simulink model "EV_Bus_Forward"  (R2025a)
settings: Solver=ode23t  StartTime=0.0  StopTime=CaseStopTime  MaxStep=Comp.MaxStep  RelTol=1e-5  AbsTol=1e-7
model workspace (MAT data in the model file):
  CaseStopTime = 300
  Comp : object (value not decoded)
  MeasuredForceBias = 1114.3044183
  MeasuredTraction = [0 0.01 0.02 0.03 0.04 0.05 0.06 0.07 0.08 0.09 0.1 0.11 ... (60002 elements, 30001x2)]
  P : object (value not decoded)
  SignalNames : object (value not decoded)
  SlopeProfile = [0 85 100 140 155 180 200 300 0 0 4 4 ... (16 elements, 8x2)]
  SpeedProfile = [0 5 25 55 70 85 105 140 160 180 200 225 ... (32 elements, 16x2)]
  TemperatureProfile = [0  25; 150  30; 300  35]
values from neighbouring files (symbols this model uses):
  Comp = struct('Tau',baseTau,'Limit',min(0.03*P.Mass*P.Gravity,0.25*driveForce),      'InitialForce',0,'Enable',1,'MinAdaptSpeed',opt(options,'MinAdaptSpeed_mps',0.5),      'MeasurementStart',0,'MeasurementEnd',duration)    [run_EV_Bus_case.m]
  P = getVariable(mw,'P')    [run_EV_Bus_case.m]
(part 2 of 2)

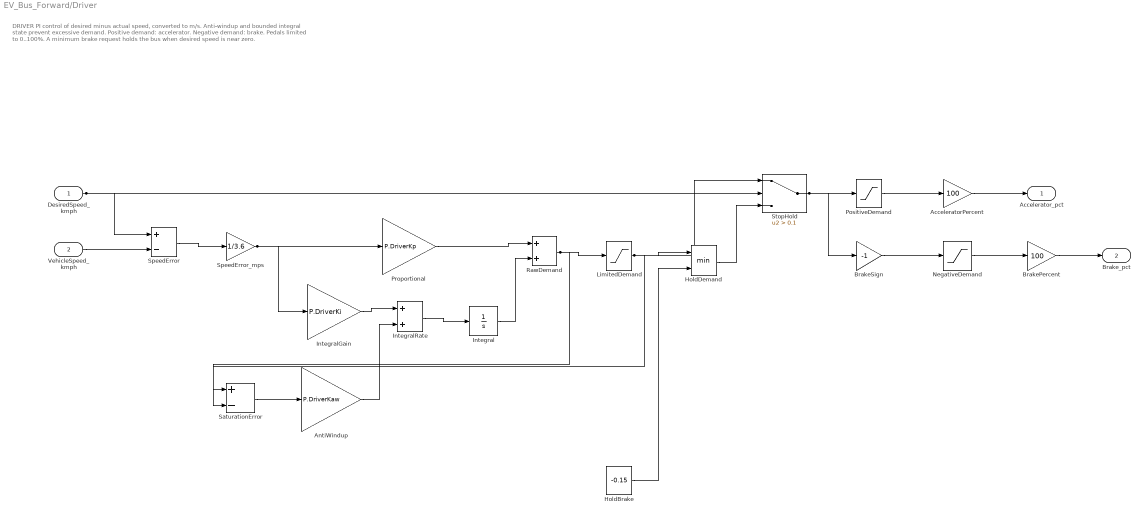
== system EV_Bus_Forward/Driver ==
  note: DRIVER
      | PI control of desired minus actual speed, converted to m/s.
      | Anti-windup and bounded integral state prevent excessive demand.
      | Positive demand: accelerator. Negative demand: brake. Pedals limited to 0..100%.
      | A minimum brake request holds the bus when desired speed is near zero.
  DesiredSpeed_kmph : Inport
  VehicleSpeed_kmph : Inport  Port=2
  AcceleratorPercent : Gain  Gain=100
  AntiWindup : Gain  Gain=P.DriverKaw
  BrakePercent : Gain  Gain=100
  BrakeSign : Gain  Gain=-1
  HoldBrake : Constant  Value=-0.15
  HoldDemand : MinMax  Inputs=2
  Integral : Integrator  LimitOutput=on  UpperSaturationLimit=0.6  LowerSaturationLimit=-0.6
  IntegralGain : Gain  Gain=P.DriverKi
  IntegralRate : Sum
  LimitedDemand : Saturate  UpperLimit=1  LowerLimit=-1
  NegativeDemand : Saturate  UpperLimit=1  LowerLimit=0
  PositiveDemand : Saturate  UpperLimit=1  LowerLimit=0
  Proportional : Gain  Gain=P.DriverKp
  RawDemand : Sum
  SaturationError : Sum  Inputs=+-
  SpeedError : Sum  Inputs=+-
  SpeedError_mps : Gain  Gain=1/3.6
  StopHold : Switch  Criteria=u2 > Threshold  Threshold=0.1  SaturateOnIntegerOverflow=off  InputSameDT=off
  Accelerator_pct : Outport
  Brake_pct : Outport  Port=2
  wires:
  AntiWindup/1 -> IntegralRate/2
  DesiredSpeed_kmph/1 -> StopHold/2, SpeedError/1
  VehicleSpeed_kmph/1 -> SpeedError/2
  RawDemand/1 -> SaturationError/2, LimitedDemand/1
  SaturationError/1 -> AntiWindup/1
  SpeedError_mps/1 -> Proportional/1, IntegralGain/1
  NegativeDemand/1 -> BrakePercent/1
  StopHold/1 -> PositiveDemand/1, BrakeSign/1
  IntegralRate/1 -> Integral/1
  SpeedError/1 -> SpeedError_mps/1
  Proportional/1 -> RawDemand/1
  IntegralGain/1 -> IntegralRate/1
  Integral/1 -> RawDemand/2
  LimitedDemand/1 -> SaturationError/1, StopHold/1, HoldDemand/1
  HoldBrake/1 -> HoldDemand/2
  HoldDemand/1 -> StopHold/3
  PositiveDemand/1 -> AcceleratorPercent/1
  BrakeSign/1 -> NegativeDemand/1
  AcceleratorPercent/1 -> Accelerator_pct/1
  BrakePercent/1 -> Brake_pct/1

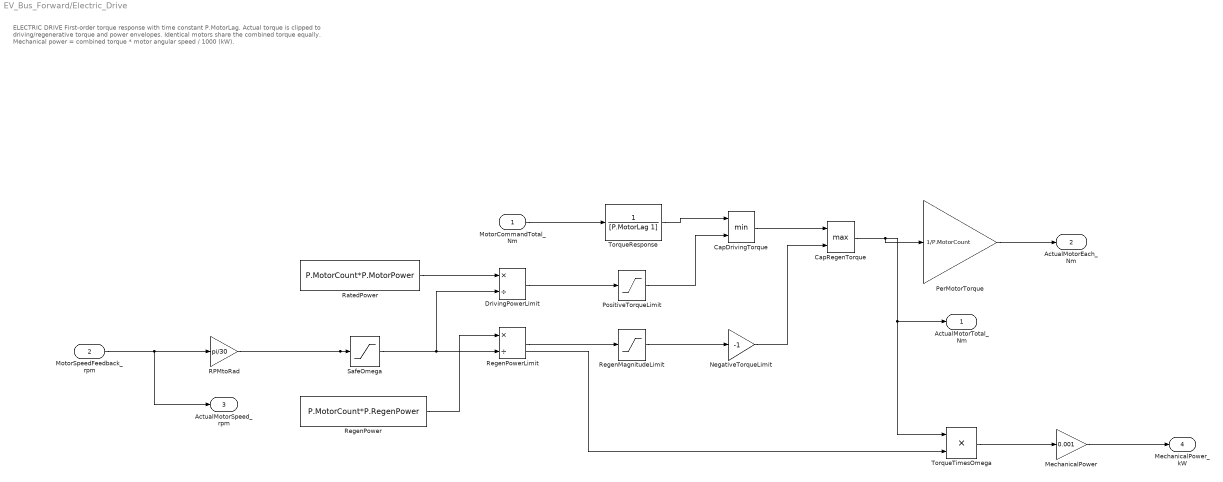
== system EV_Bus_Forward/Electric_Drive ==
  note: ELECTRIC DRIVE
      | First-order torque response with time constant P.MotorLag.
      | Actual torque is clipped to driving/regenerative torque and power envelopes.
      | Identical motors share the combined torque equally.
      | Mechanical power = combined torque * motor angular speed / 1000 (kW).
  MotorCommandTotal_Nm : Inport
  MotorSpeedFeedback_rpm : Inport  Port=2
  CapDrivingTorque : MinMax  Inputs=2
  CapRegenTorque : MinMax  Function=max  Inputs=2
  DrivingPowerLimit : Product  Inputs=*/
  MechanicalPower : Gain  Gain=0.001
  NegativeTorqueLimit : Gain  Gain=-1
  PerMotorTorque : Gain  Gain=1/P.MotorCount
  PositiveTorqueLimit : Saturate  UpperLimit=P.MotorCount*P.MotorPeakTorque  LowerLimit=0
  RPMtoRad : Gain  Gain=pi/30
  RatedPower : Constant  Value=P.MotorCount*P.MotorPower
  RegenMagnitudeLimit : Saturate  UpperLimit=P.MotorCount*P.RegenPeakTorque  LowerLimit=0
  RegenPower : Constant  Value=P.MotorCount*P.RegenPower
  RegenPowerLimit : Product  Inputs=*/
  SafeOmega : Saturate  UpperLimit=inf  LowerLimit=1
  TorqueResponse : TransferFcn  Denominator=[P.MotorLag 1]
  TorqueTimesOmega : Product  Inputs=**
  ActualMotorTotal_Nm : Outport
  ActualMotorEach_Nm : Outport  Port=2
  ActualMotorSpeed_rpm : Outport  Port=3
  MechanicalPower_kW : Outport  Port=4
  wires:
  MotorCommandTotal_Nm/1 -> TorqueResponse/1
  SafeOmega/1 -> RegenPowerLimit/2, DrivingPowerLimit/2
  MotorSpeedFeedback_rpm/1 -> ActualMotorSpeed_rpm/1, RPMtoRad/1
  RegenPower/1 -> RegenPowerLimit/1
  RegenPowerLimit/1 -> RegenMagnitudeLimit/1
  DrivingPowerLimit/1 -> PositiveTorqueLimit/1
  RatedPower/1 -> DrivingPowerLimit/1
  RPMtoRad/1 -> TorqueTimesOmega/2, SafeOmega/1
  TorqueTimesOmega/1 -> MechanicalPower/1
  TorqueResponse/1 -> CapDrivingTorque/1
  RegenMagnitudeLimit/1 -> NegativeTorqueLimit/1
  PositiveTorqueLimit/1 -> CapDrivingTorque/2
  CapDrivingTorque/1 -> CapRegenTorque/1
  NegativeTorqueLimit/1 -> CapRegenTorque/2
  MechanicalPower/1 -> MechanicalPower_kW/1
  CapRegenTorque/1 -> TorqueTimesOmega/1, ActualMotorTotal_Nm/1, PerMotorTorque/1
  PerMotorTorque/1 -> ActualMotorEach_Nm/1

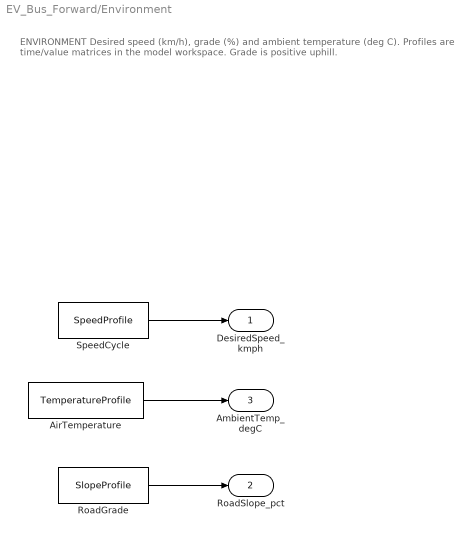
== system EV_Bus_Forward/Environment ==
  note: ENVIRONMENT
      | Desired speed (km/h), grade (%) and ambient temperature (deg C).
      | Profiles are time/value matrices in the model workspace. Grade is positive uphill.
  AirTemperature : FromWorkspace  VariableName=TemperatureProfile
  RoadGrade : FromWorkspace  VariableName=SlopeProfile
  SpeedCycle : FromWorkspace  VariableName=SpeedProfile
  DesiredSpeed_kmph : Outport
  RoadSlope_pct : Outport  Port=2
  AmbientTemp_degC : Outport  Port=3
  wires:
  RoadGrade/1 -> RoadSlope_pct/1
  AirTemperature/1 -> AmbientTemp_degC/1
  SpeedCycle/1 -> DesiredSpeed_kmph/1

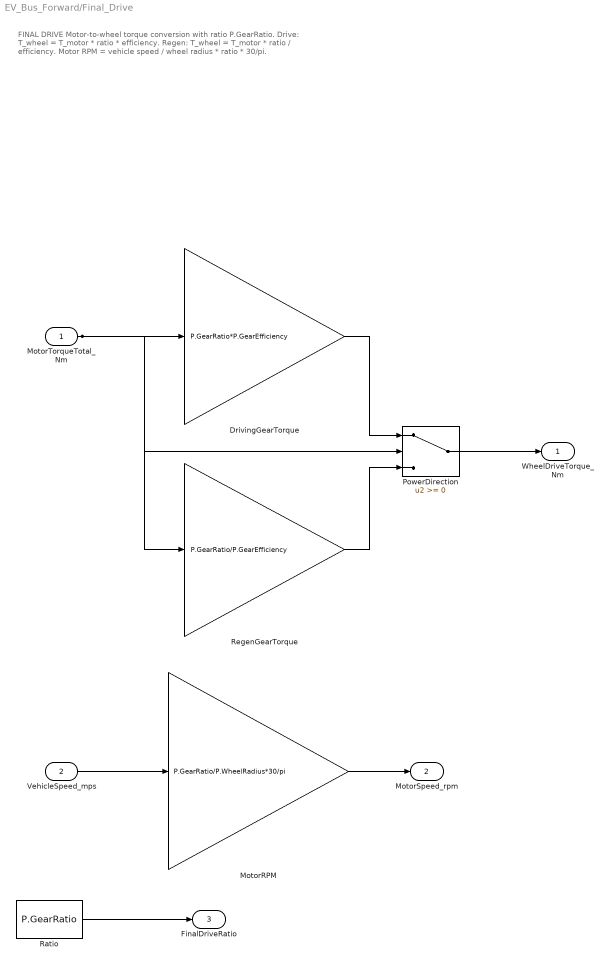
== system EV_Bus_Forward/Final_Drive ==
  note: FINAL DRIVE
      | Motor-to-wheel torque conversion with ratio P.GearRatio.
      | Drive: T_wheel = T_motor * ratio * efficiency.
      | Regen: T_wheel = T_motor * ratio / efficiency.
      | Motor RPM = vehicle speed / wheel radius * ratio * 30/pi.
  MotorTorqueTotal_Nm : Inport
  VehicleSpeed_mps : Inport  Port=2
  DrivingGearTorque : Gain  Gain=P.GearRatio*P.GearEfficiency
  MotorRPM : Gain  Gain=P.GearRatio/P.WheelRadius*30/pi
  PowerDirection : Switch  SaturateOnIntegerOverflow=off  InputSameDT=off
  Ratio : Constant  Value=P.GearRatio
  RegenGearTorque : Gain  Gain=P.GearRatio/P.GearEfficiency
  WheelDriveTorque_Nm : Outport
  MotorSpeed_rpm : Outport  Port=2
  FinalDriveRatio : Outport  Port=3
  wires:
  MotorTorqueTotal_Nm/1 -> PowerDirection/2, RegenGearTorque/1, DrivingGearTorque/1
  PowerDirection/1 -> WheelDriveTorque_Nm/1
  MotorRPM/1 -> MotorSpeed_rpm/1
  RegenGearTorque/1 -> PowerDirection/3
  DrivingGearTorque/1 -> PowerDirection/1
  Ratio/1 -> FinalDriveRatio/1
  VehicleSpeed_mps/1 -> MotorRPM/1

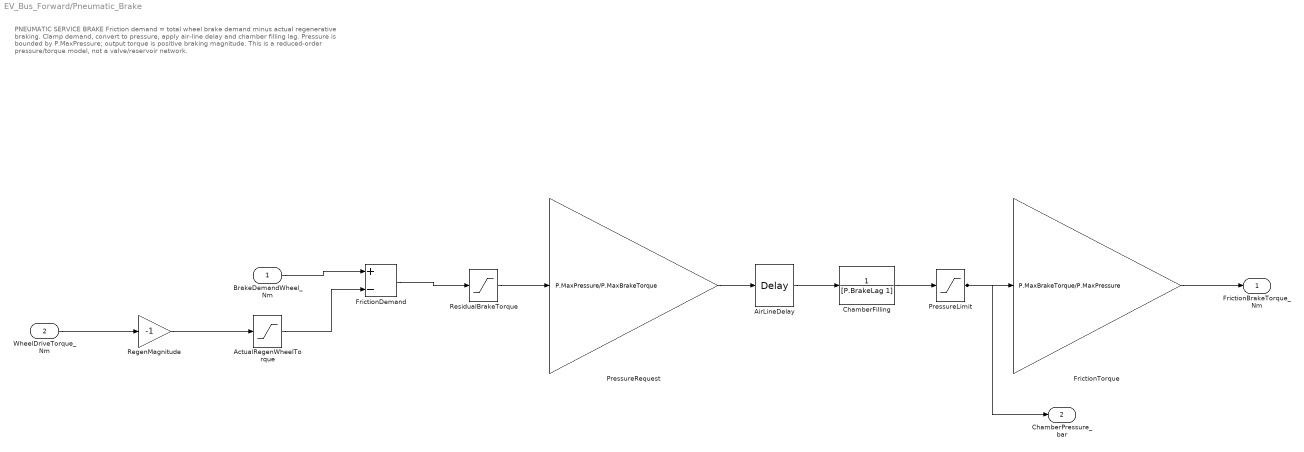
== system EV_Bus_Forward/Pneumatic_Brake ==
  note: PNEUMATIC SERVICE BRAKE
      | Friction demand = total wheel brake demand minus actual regenerative braking.
      | Clamp demand, convert to pressure, apply air-line delay and chamber filling lag.
      | Pressure is bounded by P.MaxPressure; output torque is positive braking magnitude.
      | This is a reduced-order pressure/torque model, not a valve/reservoir network.
  BrakeDemandWheel_Nm : Inport
  WheelDriveTorque_Nm : Inport  Port=2
  ActualRegenWheelTorque : Saturate  UpperLimit=inf  LowerLimit=0
  AirLineDelay : TransportDelay  DelayTime=P.BrakeDelay
  ChamberFilling : TransferFcn  Denominator=[P.BrakeLag 1]
  FrictionDemand : Sum  Inputs=+-
  FrictionTorque : Gain  Gain=P.MaxBrakeTorque/P.MaxPressure
  PressureLimit : Saturate  UpperLimit=P.MaxPressure  LowerLimit=0
  PressureRequest : Gain  Gain=P.MaxPressure/P.MaxBrakeTorque
  RegenMagnitude : Gain  Gain=-1
  ResidualBrakeTorque : Saturate  UpperLimit=P.MaxBrakeTorque  LowerLimit=0
  FrictionBrakeTorque_Nm : Outport
  ChamberPressure_bar : Outport  Port=2
  wires:
  BrakeDemandWheel_Nm/1 -> FrictionDemand/1
  AirLineDelay/1 -> ChamberFilling/1
  FrictionDemand/1 -> ResidualBrakeTorque/1
  PressureLimit/1 -> ChamberPressure_bar/1, FrictionTorque/1
  ActualRegenWheelTorque/1 -> FrictionDemand/2
  FrictionTorque/1 -> FrictionBrakeTorque_Nm/1
  WheelDriveTorque_Nm/1 -> RegenMagnitude/1
  PressureRequest/1 -> AirLineDelay/1
  ResidualBrakeTorque/1 -> PressureRequest/1
  RegenMagnitude/1 -> ActualRegenWheelTorque/1
  ChamberFilling/1 -> PressureLimit/1

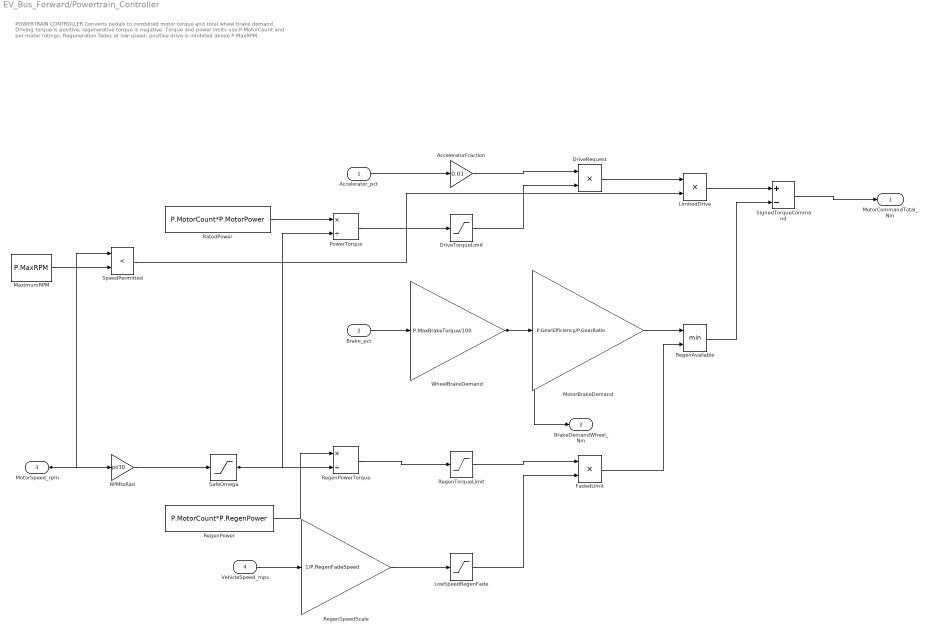
== system EV_Bus_Forward/Powertrain_Controller ==
  note: POWERTRAIN CONTROLLER
      | Converts pedals to combined motor torque and total wheel brake demand.
      | Driving torque is positive; regenerative torque is negative.
      | Torque and power limits use P.MotorCount and per-motor ratings.
      | Regeneration fades at low speed; positive drive is inhibited above P.MaxRPM.
  Accelerator_pct : Inport
  Brake_pct : Inport  Port=2
  MotorSpeed_rpm : Inport  Port=3
  VehicleSpeed_mps : Inport  Port=4
  AcceleratorFraction : Gain  Gain=0.01
  DriveRequest : Product  Inputs=**
  DriveTorqueLimit : Saturate  UpperLimit=P.MotorCount*P.MotorPeakTorque  LowerLimit=0
  FadedLimit : Product  Inputs=**
  LimitedDrive : Product  Inputs=**
  LowSpeedRegenFade : Saturate  UpperLimit=1  LowerLimit=0
  MaximumRPM : Constant  Value=P.MaxRPM
  MotorBrakeDemand : Gain  Gain=P.GearEfficiency/P.GearRatio
  PowerTorque : Product  Inputs=*/
  RPMtoRad : Gain  Gain=pi/30
  RatedPower : Constant  Value=P.MotorCount*P.MotorPower
  RegenAvailable : MinMax  Inputs=2
  RegenPower : Constant  Value=P.MotorCount*P.RegenPower
  RegenPowerTorque : Product  Inputs=*/
  RegenSpeedScale : Gain  Gain=1/P.RegenFadeSpeed
  RegenTorqueLimit : Saturate  UpperLimit=P.MotorCount*P.RegenPeakTorque  LowerLimit=0
  SafeOmega : Saturate  UpperLimit=inf  LowerLimit=1
  SignedTorqueCommand : Sum  Inputs=+-
  SpeedPermitted : RelationalOperator  Operator=<  OutDataTypeStr=boolean  RndMeth=Simplest  InputSameDT=off
  WheelBrakeDemand : Gain  Gain=P.MaxBrakeTorque/100
  MotorCommandTotal_Nm : Outport
  BrakeDemandWheel_Nm : Outport  Port=2
  wires:
  VehicleSpeed_mps/1 -> RegenSpeedScale/1
  FadedLimit/1 -> RegenAvailable/2
  MotorSpeed_rpm/1 -> SpeedPermitted/1, RPMtoRad/1
  DriveRequest/1 -> LimitedDrive/1
  MaximumRPM/1 -> SpeedPermitted/2
  SpeedPermitted/1 -> LimitedDrive/2
  RPMtoRad/1 -> SafeOmega/1
  RegenPower/1 -> RegenPowerTorque/1
  RegenAvailable/1 -> SignedTorqueCommand/2
  PowerTorque/1 -> DriveTorqueLimit/1
  SafeOmega/1 -> RegenPowerTorque/2, PowerTorque/2
  RegenTorqueLimit/1 -> FadedLimit/1
  RatedPower/1 -> PowerTorque/1
  LimitedDrive/1 -> SignedTorqueCommand/1
  DriveTorqueLimit/1 -> DriveRequest/2
  Accelerator_pct/1 -> AcceleratorFraction/1
  Brake_pct/1 -> WheelBrakeDemand/1
  RegenPowerTorque/1 -> RegenTorqueLimit/1
  RegenSpeedScale/1 -> LowSpeedRegenFade/1
  AcceleratorFraction/1 -> DriveRequest/1
  WheelBrakeDemand/1 -> BrakeDemandWheel_Nm/1, MotorBrakeDemand/1
  LowSpeedRegenFade/1 -> FadedLimit/2
  MotorBrakeDemand/1 -> RegenAvailable/1
  SignedTorqueCommand/1 -> MotorCommandTotal_Nm/1

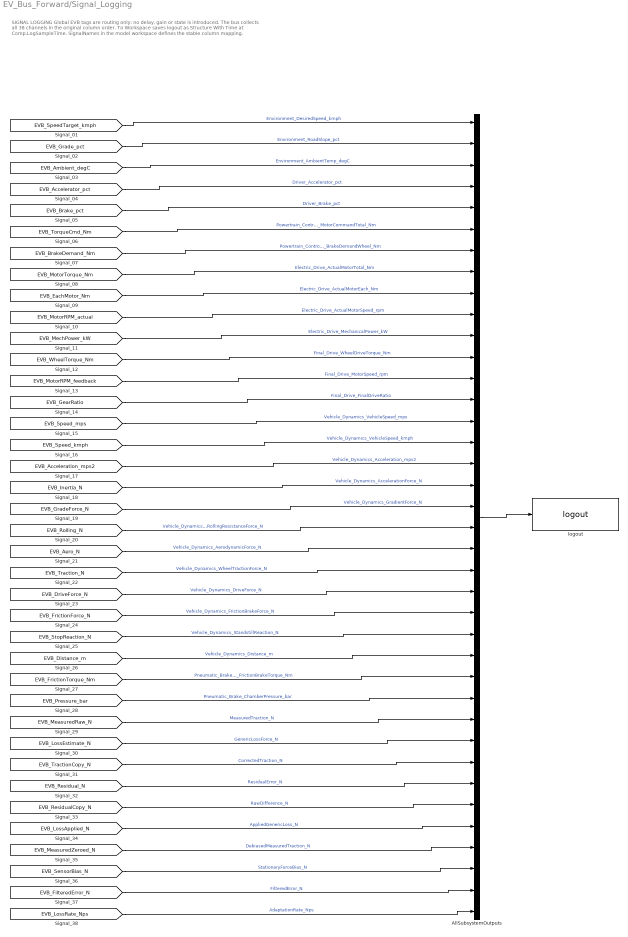
== system EV_Bus_Forward/Signal_Logging ==
  note: SIGNAL LOGGING
      | Global EVB tags are routing only: no delay, gain or state is introduced.
      | The bus collects all 38 channels in the original column order.
      | To Workspace saves logout as Structure With Time at Comp.LogSampleTime.
      | SignalNames in the model workspace defines the stable column mapping.
  AllSubsystemOutputs : BusCreator  Inputs=38
  logout : ToWorkspace  VariableName=logout  SaveFormat=Structure With Time  SampleTime=Comp.LogSampleTime
  wires:
  [EVB_LossRate_Nps] -> AllSubsystemOutputs/38  "AdaptationRate_Nps"
  [EVB_FilteredError_N] -> AllSubsystemOutputs/37  "FilteredError_N"
  [EVB_SensorBias_N] -> AllSubsystemOutputs/36  "StationaryForceBias_N"
  [EVB_MeasuredZeroed_N] -> AllSubsystemOutputs/35  "DebiasedMeasuredTraction_N"
  [EVB_LossApplied_N] -> AllSubsystemOutputs/34  "AppliedGenericLoss_N"
  [EVB_ResidualCopy_N] -> AllSubsystemOutputs/33  "RawDifference_N"
  [EVB_Residual_N] -> AllSubsystemOutputs/32  "ResidualError_N"
  [EVB_TractionCopy_N] -> AllSubsystemOutputs/31  "CorrectedTraction_N"
  [EVB_LossEstimate_N] -> AllSubsystemOutputs/30  "GenericLossForce_N"
  [EVB_MeasuredRaw_N] -> AllSubsystemOutputs/29  "MeasuredTraction_N"
  [EVB_Pressure_bar] -> AllSubsystemOutputs/28  "Pneumatic_Brake_ChamberPressure_bar"
  [EVB_FrictionTorque_Nm] -> AllSubsystemOutputs/27  "Pneumatic_Brake_FrictionBrakeTorque_Nm"
  [EVB_Distance_m] -> AllSubsystemOutputs/26  "Vehicle_Dynamics_Distance_m"
  [EVB_StopReaction_N] -> AllSubsystemOutputs/25  "Vehicle_Dynamics_StandstillReaction_N"
  [EVB_FrictionForce_N] -> AllSubsystemOutputs/24  "Vehicle_Dynamics_FrictionBrakeForce_N"
  [EVB_DriveForce_N] -> AllSubsystemOutputs/23  "Vehicle_Dynamics_DriveForce_N"
  [EVB_Traction_N] -> AllSubsystemOutputs/22  "Vehicle_Dynamics_WheelTractionForce_N"
  [EVB_Aero_N] -> AllSubsystemOutputs/21  "Vehicle_Dynamics_AerodynamicForce_N"
  [EVB_Rolling_N] -> AllSubsystemOutputs/20  "Vehicle_Dynamics_RollingResistanceForce_N"
  [EVB_GradeForce_N] -> AllSubsystemOutputs/19  "Vehicle_Dynamics_GradientForce_N"
  [EVB_Inertia_N] -> AllSubsystemOutputs/18  "Vehicle_Dynamics_AccelerationForce_N"
  [EVB_Acceleration_mps2] -> AllSubsystemOutputs/17  "Vehicle_Dynamics_Acceleration_mps2"
  [EVB_Speed_kmph] -> AllSubsystemOutputs/16  "Vehicle_Dynamics_VehicleSpeed_kmph"
  [EVB_Speed_mps] -> AllSubsystemOutputs/15  "Vehicle_Dynamics_VehicleSpeed_mps"
  [EVB_GearRatio] -> AllSubsystemOutputs/14  "Final_Drive_FinalDriveRatio"
  [EVB_MotorRPM_feedback] -> AllSubsystemOutputs/13  "Final_Drive_MotorSpeed_rpm"
  [EVB_WheelTorque_Nm] -> AllSubsystemOutputs/12  "Final_Drive_WheelDriveTorque_Nm"
  [EVB_MechPower_kW] -> AllSubsystemOutputs/11  "Electric_Drive_MechanicalPower_kW"
  [EVB_MotorRPM_actual] -> AllSubsystemOutputs/10  "Electric_Drive_ActualMotorSpeed_rpm"
  [EVB_EachMotor_Nm] -> AllSubsystemOutputs/9  "Electric_Drive_ActualMotorEach_Nm"
  [EVB_MotorTorque_Nm] -> AllSubsystemOutputs/8  "Electric_Drive_ActualMotorTotal_Nm"
  [EVB_BrakeDemand_Nm] -> AllSubsystemOutputs/7  "Powertrain_Controller_BrakeDemandWheel_Nm"
  [EVB_TorqueCmd_Nm] -> AllSubsystemOutputs/6  "Powertrain_Controller_MotorCommandTotal_Nm"
  [EVB_Brake_pct] -> AllSubsystemOutputs/5  "Driver_Brake_pct"
  [EVB_Accelerator_pct] -> AllSubsystemOutputs/4  "Driver_Accelerator_pct"
  [EVB_Ambient_degC] -> AllSubsystemOutputs/3  "Environment_AmbientTemp_degC"
  [EVB_Grade_pct] -> AllSubsystemOutputs/2  "Environment_RoadSlope_pct"
  [EVB_SpeedTarget_kmph] -> AllSubsystemOutputs/1  "Environment_DesiredSpeed_kmph"
  AllSubsystemOutputs/1 -> logout/1

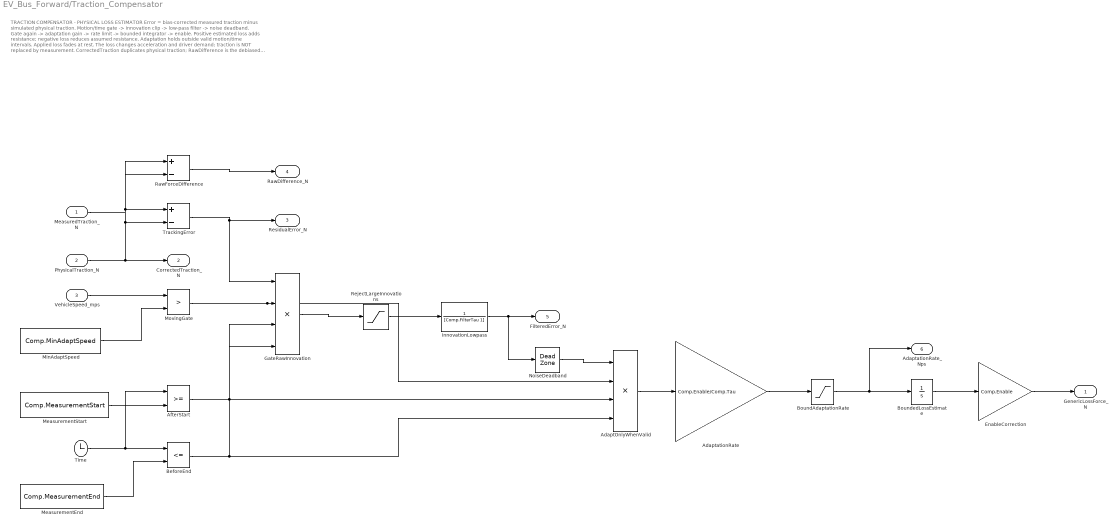
== system EV_Bus_Forward/Traction_Compensator ==
  note: TRACTION COMPENSATOR - PHYSICAL LOSS ESTIMATOR
      | Error = bias-corrected measured traction minus simulated physical traction.
      | Motion/time gate -> innovation clip -> low-pass filter -> noise deadband.
      | Gate again -> adaptation gain -> rate limit -> bounded integrator -> enable.
      | Positive estimated loss adds resistance; negative loss reduces assumed resistance.
      | Adaptation holds outside valid motion/time intervals. Applied loss fades at rest.
      | The loss changes acceleration and driver demand; traction is NOT replaced by measurement.
      | CorrectedTraction duplicates physical traction; RawDifference is the debiased residual.
  MeasuredTraction_N : Inport
  PhysicalTraction_N : Inport  Port=2
  VehicleSpeed_mps : Inport  Port=3
  AdaptOnlyWhenValid : Product  Inputs=****
  AdaptationRate : Gain  Gain=Comp.Enable/Comp.Tau
  AfterStart : RelationalOperator  OutDataTypeStr=boolean  RndMeth=Simplest  InputSameDT=off
  BeforeEnd : RelationalOperator  Operator=<=  OutDataTypeStr=boolean  RndMeth=Simplest  InputSameDT=off
  BoundAdaptationRate : Saturate  UpperLimit=Comp.MaxRate  LowerLimit=-Comp.MaxRate
  BoundedLossEstimate : Integrator  InitialCondition=Comp.InitialForce  LimitOutput=on  UpperSaturationLimit=Comp.Limit  LowerSaturationLimit=-Comp.Limit
  EnableCorrection : Gain  Gain=Comp.Enable
  GateRawInnovation : Product  Inputs=****
  InnovationLowpass : TransferFcn  Denominator=[Comp.FilterTau 1]
  MeasurementEnd : Constant  Value=Comp.MeasurementEnd
  MeasurementStart : Constant  Value=Comp.MeasurementStart
  MinAdaptSpeed : Constant  Value=Comp.MinAdaptSpeed
  MovingGate : RelationalOperator  Operator=>  OutDataTypeStr=boolean  RndMeth=Simplest  InputSameDT=off
  NoiseDeadband : DeadZone  LowerValue=-Comp.Deadband  UpperValue=Comp.Deadband
  RawForceDifference : Sum  Inputs=+-
  RejectLargeInnovations : Saturate  UpperLimit=Comp.ErrorClip  LowerLimit=-Comp.ErrorClip
  Time : Clock
  TrackingError : Sum  Inputs=+-
  GenericLossForce_N : Outport
  CorrectedTraction_N : Outport  Port=2
  ResidualError_N : Outport  Port=3
  RawDifference_N : Outport  Port=4
  FilteredError_N : Outport  Port=5
  AdaptationRate_Nps : Outport  Port=6
  wires:
  PhysicalTraction_N/1 -> RawForceDifference/2, TrackingError/2, CorrectedTraction_N/1
  MeasuredTraction_N/1 -> RawForceDifference/1, TrackingError/1
  VehicleSpeed_mps/1 -> MovingGate/1
  RawForceDifference/1 -> RawDifference_N/1
  MovingGate/1 -> AdaptOnlyWhenValid/2, GateRawInnovation/2
  TrackingError/1 -> GateRawInnovation/1, ResidualError_N/1
  MeasurementEnd/1 -> BeforeEnd/2
  MinAdaptSpeed/1 -> MovingGate/2
  Time/1 -> BeforeEnd/1, AfterStart/1
  RejectLargeInnovations/1 -> InnovationLowpass/1
  MeasurementStart/1 -> AfterStart/2
  AfterStart/1 -> AdaptOnlyWhenValid/3, GateRawInnovation/3
  AdaptationRate/1 -> BoundAdaptationRate/1
  BeforeEnd/1 -> GateRawInnovation/4, AdaptOnlyWhenValid/4
  GateRawInnovation/1 -> RejectLargeInnovations/1
  InnovationLowpass/1 -> NoiseDeadband/1, FilteredError_N/1
  NoiseDeadband/1 -> AdaptOnlyWhenValid/1
  BoundAdaptationRate/1 -> AdaptationRate_Nps/1, BoundedLossEstimate/1
  AdaptOnlyWhenValid/1 -> AdaptationRate/1
  BoundedLossEstimate/1 -> EnableCorrection/1
  EnableCorrection/1 -> GenericLossForce_N/1

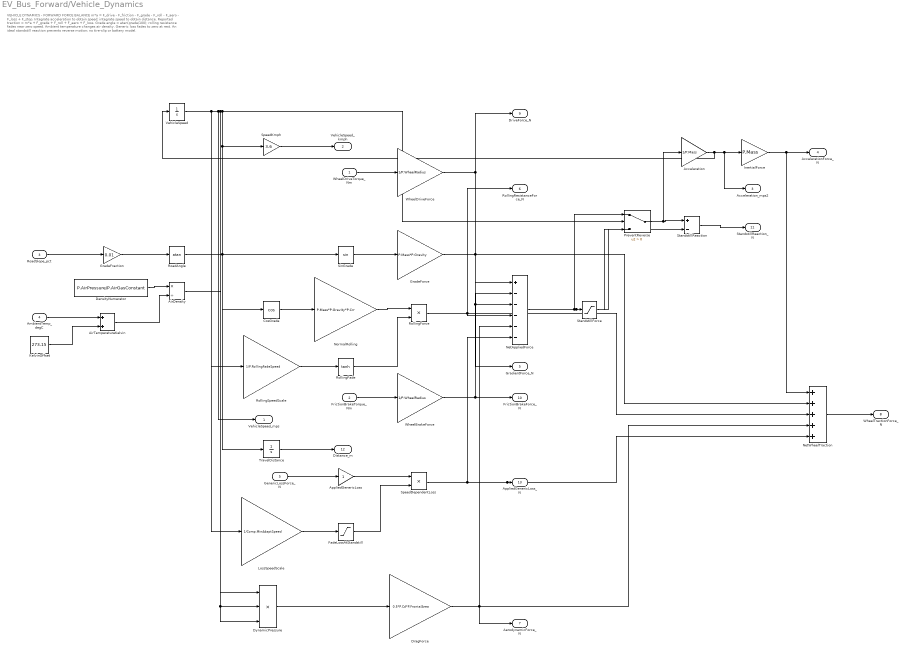
== system EV_Bus_Forward/Vehicle_Dynamics ==
  note: VEHICLE DYNAMICS - FORWARD FORCE BALANCE
      | m*a = F_drive - F_friction - F_grade - F_roll - F_aero - F_loss + F_stop.
      | Integrate acceleration to obtain speed; integrate speed to obtain distance.
      | Reported traction = m*a + F_grade + F_roll + F_aero + F_loss.
      | Grade angle = atan(grade/100); rolling resistance fades near zero speed.
      | Ambient temperature changes air density. Generic loss fades to zero at rest.
      | An ideal standstill reaction prevents reverse motion; no tire-slip or battery model.
  WheelDriveTorque_Nm : Inport
  FrictionBrakeTorque_Nm : Inport  Port=2
  RoadSlope_pct : Inport  Port=3
  AmbientTemp_degC : Inport  Port=4
  GenericLossForce_N : Inport  Port=5
  Acceleration : Gain  Gain=1/P.Mass
  AirDensity : Product  Inputs=*/
  AirTemperatureKelvin : Sum
  AppliedGenericLoss : Gain
  CosGrade : Trigonometry  Operator=cos
  DensityNumerator : Constant  Value=P.AirPressure/P.AirGasConstant
  DragForce : Gain  Gain=0.5*P.Cd*P.FrontalArea
  DynamicPressure : Product  Inputs=***
  FadeLossAtStandstill : Saturate  UpperLimit=1  LowerLimit=0
  GradeForce : Gain  Gain=P.Mass*P.Gravity
  GradeFraction : Gain  Gain=0.01
  InertialForce : Gain  Gain=P.Mass
  KelvinOffset : Constant  Value=273.15
  LossSpeedScale : Gain  Gain=1/Comp.MinAdaptSpeed
  NetAppliedForce : Sum  Inputs=+-----
  NetWheelTraction : Sum  Inputs=+++++
  NormalRolling : Gain  Gain=P.Mass*P.Gravity*P.Crr
  PreventReverse : Switch  Criteria=u2 > Threshold  SaturateOnIntegerOverflow=off  InputSameDT=off
  RoadAngle : Trigonometry  Operator=atan
  RollingFade : Trigonometry  Operator=tanh
  RollingForce : Product  Inputs=**
  RollingSpeedScale : Gain  Gain=1/P.RollingFadeSpeed
  SinGrade : Trigonometry
  SpeedDependentLoss : Product  Inputs=**
  SpeedKmph : Gain  Gain=3.6
  StandstillForce : Saturate  UpperLimit=inf  LowerLimit=0
  StandstillReaction : Sum  Inputs=+-
  TravelDistance : Integrator
  VehicleSpeed : Integrator  InitialCondition=P.InitialSpeed  LimitOutput=on  LowerSaturationLimit=0
  WheelBrakeForce : Gain  Gain=1/P.WheelRadius
  WheelDriveForce : Gain  Gain=1/P.WheelRadius
  VehicleSpeed_mps : Outport
  VehicleSpeed_kmph : Outport  Port=2
  Acceleration_mps2 : Outport  Port=3
  AccelerationForce_N : Outport  Port=4
  GradientForce_N : Outport  Port=5
  RollingResistanceForce_N : Outport  Port=6
  AerodynamicForce_N : Outport  Port=7
  WheelTractionForce_N : Outport  Port=8
  DriveForce_N : Outport  Port=9
  FrictionBrakeForce_N : Outport  Port=10
  StandstillReaction_N : Outport  Port=11
  Distance_m : Outport  Port=12
  AppliedGenericLoss_N : Outport  Port=13
  wires:
  Acceleration/1 -> InertialForce/1, Acceleration_mps2/1, VehicleSpeed/1
  AirTemperatureKelvin/1 -> AirDensity/2
  AppliedGenericLoss/1 -> SpeedDependentLoss/1
  AmbientTemp_degC/1 -> AirTemperatureKelvin/1
  RoadSlope_pct/1 -> GradeFraction/1
  DensityNumerator/1 -> AirDensity/1
  LossSpeedScale/1 -> FadeLossAtStandstill/1
  GradeFraction/1 -> RoadAngle/1
  GradeForce/1 -> NetAppliedForce/3, GradientForce_N/1, NetWheelTraction/2
  CosGrade/1 -> NormalRolling/1
  KelvinOffset/1 -> AirTemperatureKelvin/2
  SpeedDependentLoss/1 -> NetWheelTraction/5, AppliedGenericLoss_N/1, NetAppliedForce/6
  VehicleSpeed/1 -> DynamicPressure/2, DynamicPressure/3, TravelDistance/1, SpeedKmph/1, PreventReverse/2, VehicleSpeed_mps/1, RollingSpeedScale/1, LossSpeedScale/1
  NormalRolling/1 -> RollingForce/1
  RoadAngle/1 -> CosGrade/1, SinGrade/1
  AirDensity/1 -> DynamicPressure/1
  WheelBrakeForce/1 -> FrictionBrakeForce_N/1, NetAppliedForce/2
  SpeedKmph/1 -> VehicleSpeed_kmph/1
  RollingSpeedScale/1 -> RollingFade/1
  TravelDistance/1 -> Distance_m/1
  WheelDriveTorque_Nm/1 -> WheelDriveForce/1
  GenericLossForce_N/1 -> AppliedGenericLoss/1
  DynamicPressure/1 -> DragForce/1
  SinGrade/1 -> GradeForce/1
  RollingFade/1 -> RollingForce/2
  FrictionBrakeTorque_Nm/1 -> WheelBrakeForce/1
  DragForce/1 -> NetWheelTraction/4, AerodynamicForce_N/1, NetAppliedForce/5
  FadeLossAtStandstill/1 -> SpeedDependentLoss/2
  StandstillForce/1 -> PreventReverse/3
  WheelDriveForce/1 -> DriveForce_N/1, NetAppliedForce/1
  RollingForce/1 -> NetWheelTraction/3, RollingResistanceForce_N/1, NetAppliedForce/4
  NetWheelTraction/1 -> WheelTractionForce_N/1
  NetAppliedForce/1 -> StandstillReaction/2, StandstillForce/1, PreventReverse/1
  PreventReverse/1 -> Acceleration/1, StandstillReaction/1
  StandstillReaction/1 -> StandstillReaction_N/1
  InertialForce/1 -> NetWheelTraction/1, AccelerationForce_N/1
